simulink model "hrg_split_reference_replay"  (R2025a)
settings: Solver=FixedStepDiscrete  StartTime=0.0  StopTime=(size(replayData,1)-1)*frameDt  FixedStep=frameDt  RelTol=1e-3
model workspace (MAT data in the model file):
  frameDt = 0.000588235294118
  replayData = [0 0.000588235294118 0.00117647058824 0.00176470588235 0.00235294117647 0.00294117647059 0.00352941176471 0.00411764705882 0.00470588235294 0.00529411764706 0.00588235294118 0.00647058823529 ... (238000 elements, 34000x7)]
  weights = [2.5445224849e-17  -2.15390142898e-11; 8.83576290589e-18  -4.61874630163e-06; 2.00267773948e-17  5.06063378765e-06; -3.04391213014e-17  -0.00171378351535; 4.43654869607e-14  0.000156035487054]
settings Model: Creator=Administrator  LastModifiedBy=Administrator

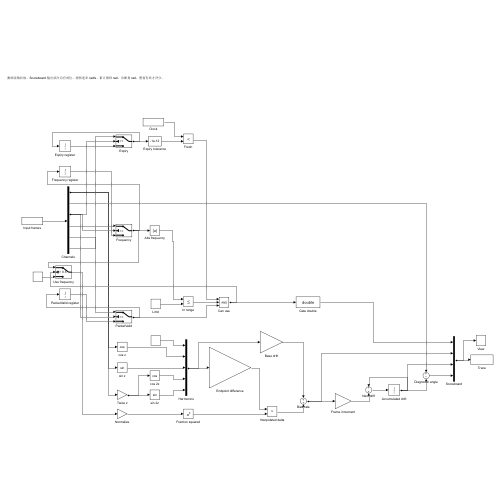
[thumbnail: Simulink's stored preview of the top-level diagram]
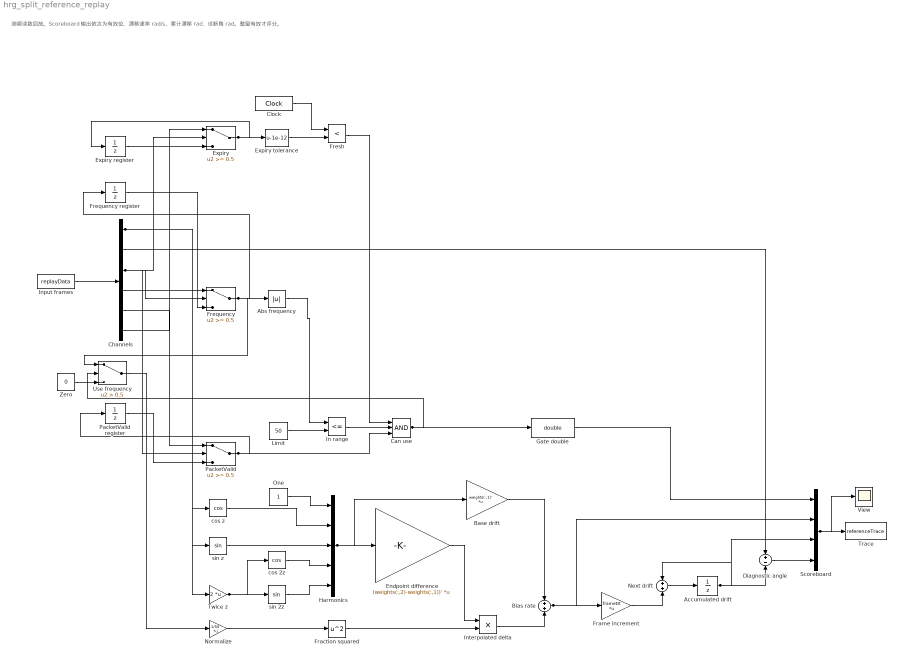
== system hrg_split_reference_replay ==
  note: 测频读数回放。Scoreboard 输出依次为有效位、漂移速率 rad/s、累计漂移 rad、诊断角 rad。整窗有效才评分。
  Abs frequency : Abs  SaturateOnIntegerOverflow=off
  Accumulated drift : UnitDelay  SampleTime=frameDt  HasFrameUpgradeWarning=on
  Base drift : Gain  Gain=weights(:,1)'  Multiplication=Matrix(K*u)
  Bias rate : Sum
  Can use : Logic  Description=包有效、未到期且频差不超过 50 mHz 时允许使用；上电和新无效包立即拒绝。  Inputs=3  AllPortsSameDT=off  OutDataTypeStr=boolean
  Channels : Demux  Description=依次为四倍驻波角、原机体角、新包事件、频差 mHz、包有效位、到期绝对时刻 s。  Outputs=6
  Clock : DigitalClock  SampleTime=frameDt
  Diagnostic angle : Sum  Description=仅整段有效区间的相对角或局部斜率可评分。跨缺口绝对角连续性未经验证。  Inputs=+-
  Endpoint difference : Gain  Gain=(weights(:,2)-weights(:,1))'  Multiplication=Matrix(K*u)
  Expiry : Switch  Threshold=0.5  SaturateOnIntegerOverflow=off  InputSameDT=off
  Expiry register : UnitDelay  SampleTime=frameDt  HasFrameUpgradeWarning=on
  Expiry tolerance : Bias  Bias=-1e-12  SaturateOnIntegerOverflow=off
  Fraction squared : Math  Operator=square
  Frame increment : Gain  Gain=frameDt  Multiplication=Matrix(K*u)
  Frequency : Switch  Threshold=0.5  SaturateOnIntegerOverflow=off  InputSameDT=off
  Frequency register : UnitDelay  SampleTime=frameDt  HasFrameUpgradeWarning=on
  Fresh : RelationalOperator  Operator=<  OutDataTypeStr=boolean  RndMeth=Simplest  InputSameDT=off
  Gate double : DataTypeConversion  OutDataTypeStr=double  SaturateOnIntegerOverflow=off  RndMeth=Floor
  Harmonics : Mux  Inputs=5
  In range : RelationalOperator  Operator=<=  OutDataTypeStr=boolean  RndMeth=Simplest  InputSameDT=off
  Input frames : FromWorkspace  VariableName=replayData  SampleTime=frameDt  Interpolate=off  OutputAfterFinalValue=Holding final value
  Interpolated delta : Product
  Limit : Constant  Value=50
  Next drift : Sum
  Normalize : Gain  Gain=1/50  Multiplication=Matrix(K*u)
  One : Constant
  PacketValid : Switch  Threshold=0.5  SaturateOnIntegerOverflow=off  InputSameDT=off
  PacketValid register : UnitDelay  SampleTime=frameDt  HasFrameUpgradeWarning=on
  Scoreboard : Mux
  Trace : ToWorkspace  VariableName=referenceTrace  SampleTime=-1
  Twice z : Gain  Gain=2  Multiplication=Matrix(K*u)
  Use frequency : Switch  Criteria=u2 > Threshold  Threshold=0.5  SaturateOnIntegerOverflow=off  InputSameDT=off
  View : Scope
  Zero : Constant  Value=0
  cos 2z : Trigonometry  Operator=cos
  cos z : Trigonometry  Operator=cos
  sin 2z : Trigonometry
  sin z : Trigonometry
  wires:
  Expiry tolerance/1 -> Fresh/2
  Input frames/1 -> Channels/1
  Zero/1 -> Use frequency/3
  Channels/3 -> Frequency/2, PacketValid/2, Expiry/2
  Expiry register/1 -> Expiry/3
  cos 2z/1 -> Harmonics/4
  Channels/2 -> Diagnostic angle/1
  Can use/1 -> Use frequency/2, Gate double/1
  Limit/1 -> In range/2
  Frequency register/1 -> Frequency/3
  Channels/1 -> cos z/1, Twice z/1, sin z/1
  Channels/4 -> Frequency/1
  Channels/5 -> PacketValid/1
  Channels/6 -> Expiry/1
  Use frequency/1 -> Normalize/1
  PacketValid register/1 -> PacketValid/3
  Expiry/1 -> Expiry register/1, Expiry tolerance/1
  Frequency/1 -> Use frequency/1, Frequency register/1, Abs frequency/1
  Accumulated drift/1 -> Next drift/1, Diagnostic angle/2, Scoreboard/3
  PacketValid/1 -> PacketValid register/1, Can use/3
  In range/1 -> Can use/2
  cos z/1 -> Harmonics/2
  Scoreboard/1 -> View/1, Trace/1
  Fraction squared/1 -> Interpolated delta/2
  sin z/1 -> Harmonics/3
  Twice z/1 -> sin 2z/1, cos 2z/1
  Normalize/1 -> Fraction squared/1
  Clock/1 -> Fresh/1
  Abs frequency/1 -> In range/1
  One/1 -> Harmonics/1
  sin 2z/1 -> Harmonics/5
  Diagnostic angle/1 -> Scoreboard/4
  Fresh/1 -> Can use/1
  Harmonics/1 -> Base drift/1, Endpoint difference/1
  Endpoint difference/1 -> Interpolated delta/1
  Base drift/1 -> Bias rate/1
  Gate double/1 -> Scoreboard/1
  Interpolated delta/1 -> Bias rate/2
  Bias rate/1 -> Scoreboard/2, Frame increment/1
  Frame increment/1 -> Next drift/2
  Next drift/1 -> Accumulated drift/1
